simulink model "QC_Physics"  (R2026b)
settings: Solver=VariableStepAuto
undefined symbols (not defined in the file): N, Nm, rad, s, X, Y, Z
libraries: nesl_utility x13, sm_lib x5, simulink x1, fl_lib x1
settings Model: Creator=dani  LastModifiedBy=Dani

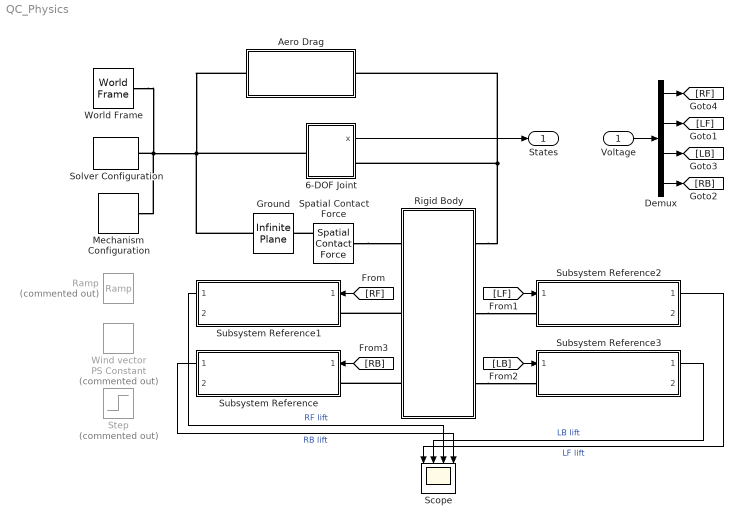
== system QC_Physics ==
  Voltage : Inport
  6-DOF Joint : Subsystem
  Aero Drag : Subsystem  ReferencedSubsystem=aero_drag
  Demux : Demux
  Ground : sm_lib/Curves and Surfaces/Infinite Plane  GraphicType=Rectangle  GraphicPlaneWidth=2  GraphicPlaneWidthUnits=m  GraphicPlaneHeight=2  GraphicPlaneHeightUnits=m  GraphicVisPropType=SimpleVisualProperties  GraphicDiffuseColor=[1 0.6667 0]  GraphicOpacity=0.4  GraphicSpecularColor=[0.5 0.5 0.5 1.0]  GraphicAmbientColor=[0.15 0.15 0.15 1.0]  GraphicEmissiveColor=[0.0 0.0 0.0 1.0]  GraphicShininess=75
  Mechanism Configuration : sm_lib/Utilities/Mechanism Configuration  UniformGravity=Constant  GravityVector=[0 0 -9.80665]  GravityVectorUnits=m/s^2  LinearizationDelta=0.001  JointModeTransitionNonlinearIterations=2
  Ramp : simulink/Sources/Ramp  Commented=on  slope=-715  start=0.37  InitialOutput=0
  Rigid Body : Subsystem  ReferencedSubsystem=rigid_body
  Scope : Scope  NumInputPorts=4
      settings: TimeSpan=1  ActiveDisplayString=4  ActiveDisplayYMinimum=-0.17596138261761787  ActiveDisplayYMaximum=1.5853977728105553  DataLoggingVariableName=ScopeData5
  Solver Configuration : nesl_utility/Solver Configuration  PhysicalDomain=network_engine_domain  SubClassName=solver  LeftPortType=input  RightPortType=generic  Tones=[]  Harmonics=[]  SimulateNoise=off  Profile=off  UseLocalSampling=off  EnableSwitchedLinearOptims=on  FrequencyDomain=off  UseCCode=off  RelTol=0.001  AbsTol=0.001  MinStep=1e-09  ToWorkspace=off  RevertToSquareIcSolve=off  NumHomotopyIterations=100  PhasorMode=off  PhasorModeNumHarmonics=1  ConsistencySolver=NEWTON_XTOL_AFTER_FTOL  CanonicalOrdering=UNORDERED  OptimizeIntermediates=UNOPTIMIZED  MulticoreSolverChoice=BACKWARD_EULER  IndexReductionMethod=DerivativeReplacement  DoDC=off  ResidualTolerance=1e-09  ConsistencyTolSource=GLOBAL  ConsistencyAbsTol=0.001  ConsistencyRelTol=0.001  ConsistencyTolFactor=0.001  UseLocalSolver=off  LocalSolverChoice=NE_BACKWARD_EULER_ADVANCER  ResolveIndetEquations=on  FunctionEvalNumThread=1  LocalSolverSampleTime=0.001  DoFixedCost=off  MaxNonlinIter=3  MaxModeIter=2  ComputeImpulses=off  ImpulseIterations=2  LinearAlgebra=auto  LinearAlgebraNumThread=0  EquationFormulation=NE_TIME_EF  DelaysMemoryBudget=1024  AutomaticFiltering=on  FilteringTimeConstant=0.001  PartitionStorageMethod=AS_NEEDED  PartitionMemoryBudget=1024  PartitionMethod=BALANCED  MultibodyUseLocalSolver=off  MultibodyLocalSolverChoice=ODE1  MultibodyLocalSolverSampleTime=0.001
  Spatial Contact Force : sm_lib/Forces and Torques/Spatial Contact Force  SenseSeparationDistance=on  NormalForceType=SmoothSpringDamper  NormalStiffness=1e3  NormalStiffnessUnits=N/m  NormalDamping=2e1  NormalDampingUnits=N/(m/s)  NormalTransitionRegionWidth=1e-3  NormalTransitionRegionWidthUnits=m  FrictionType=SmoothStickSlip  CoefficientOfStaticFriction=0.4  CoefficientOfDynamicFriction=0.4  FrictionalCriticalVelocity=1e-2  FrictionalCriticalVelocityUnits=m/s  SenseContactSignal=off  SensePenetrationDepth=off  SenseNormalVelocity=off  SenseTangentialVelocity=off  SensingForceTorqueDirection=BaseOnFollower  SensingForceTorqueResolutionFrame=ContactFrame  SenseNormalForce=off  SenseNormalForceMagnitude=off  SenseNormalTorque=off  SenseFrictionalForce=off  SenseFrictionalForceMagnitude=off  SenseFrictionalTorque=off  SenseTotalForce=off  SenseTotalTorque=off  SenseContactBaseRotation=off  SenseContactBaseTranslation=off  SenseContactFollowerRotation=off  SenseContactFollowerTranslation=off  ZeroCrossDetectContactStartAndEnd=on
  Step : Step  Commented=on  Time=2  FinalValue=4.1  SampleTime=0
  Subsystem Reference : Subsystem  ReferencedSubsystem=thruster  Dir=CCW  w2F=1e-3  w2F_u=N*s/rad  w2T=1e-5  w2T_u=Nm*s/rad  Color=[0 1 0]
  Subsystem Reference1 : Subsystem  ReferencedSubsystem=thruster  Dir=CW  w2F=1e-3  w2F_u=N*s/rad  w2T=1e-5  w2T_u=Nm*s/rad  Color=[1 0 0]
  Subsystem Reference2 : Subsystem  ReferencedSubsystem=thruster  Dir=CCW  w2F=1e-3  w2F_u=N*s/rad  w2T=1e-5  w2T_u=Nm*s/rad  Color=[0 1 0]
  Subsystem Reference3 : Subsystem  ReferencedSubsystem=thruster  Dir=CW  w2F=1e-3  w2F_u=N*s/rad  w2T=1e-5  w2T_u=Nm*s/rad  Color=[1 0 0]
  Wind vector : fl_lib/Physical Signals/Sources/PS Constant  Commented=on  constant=[1 0 0] m/s
  World Frame : sm_lib/Frames and Transforms/World Frame
  States : Outport
  wires:
  Demux/3 -> [LB]
  Demux/4 -> [RB]
  [RB] -> Subsystem Reference/1
  Subsystem Reference3/1 -> Scope/2  "LB lift"
  Subsystem Reference1/1 -> Scope/3  "RF lift"
  Voltage/1 -> Demux/1
  [LB] -> Subsystem Reference3/1
  Demux/1 -> [RF]
  [LF] -> Subsystem Reference2/1
  Subsystem Reference/1 -> Scope/4  "RB lift"
  [RF] -> Subsystem Reference1/1
  Subsystem Reference2/1 -> Scope/1  "LF lift"
  Demux/2 -> [LF]
  6-DOF Joint/1(x) -> States/1
  connections:
  6-DOF Joint/RConn1 -- Aero Drag/RConn1 -- Rigid Body/LConn1
  Solver Configuration/RConn1 -- Ground/LConn1 -- Aero Drag/LConn1 -- 6-DOF Joint/LConn1 -- World Frame/RConn1 -- Mechanism Configuration/RConn1
  Rigid Body/RConn3 -- Subsystem Reference/LConn1
  Rigid Body/LConn3 -- Subsystem Reference3/LConn1
  Spatial Contact Force/RConn1 -- Ground/RConn1
  Rigid Body/RConn2 -- Subsystem Reference1/LConn1
  Spatial Contact Force/LConn1 -- Rigid Body/RConn1
  Rigid Body/LConn2 -- Subsystem Reference2/LConn1

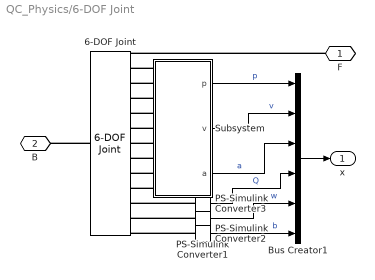
== system QC_Physics/6-DOF Joint ==
  6-DOF Joint : sm_lib/Joints/6-DOF Joint  JointMode=Normal  CompositeWrenchDir=FollowerOnBase  CompositeWrenchFrame=BaseFrame  SenseConstraintForce=off  SenseConstraintTorque=off  SenseTotalForce=off  SenseTotalTorque=off  PxPositionTargetSpecify=off  PxPositionTargetPriority=High  PxPositionTargetValue=0  PxPositionTargetValueUnits=m  PxVelocityTargetSpecify=off  PxVelocityTargetPriority=High  PxVelocityTargetValue=0  PxVelocityTargetValueUnits=m/s  PxEquilibriumPosition=0  PxEquilibriumPositionUnits=m  PxSpringStiffness=0  PxSpringStiffnessUnits=N/m  PxDampingCoefficient=0  PxDampingCoefficientUnits=N/(m/s)  PxLowerLimitSpecify=off  PxLowerLimitBound=-1  PxLowerLimitBoundUnits=m  PxLowerLimitStiffness=1e6  PxLowerLimitStiffnessUnits=N/m  PxLowerLimitDamping=1e3  PxLowerLimitDampingUnits=N/(m/s)  PxLowerLimitTransitionRegionWidth=1e-4  PxLowerLimitTransitionRegionWidthUnits=m  PxUpperLimitSpecify=off  PxUpperLimitBound=1  PxUpperLimitBoundUnits=m  PxUpperLimitStiffness=1e6  PxUpperLimitStiffnessUnits=N/m  PxUpperLimitDamping=1e3  PxUpperLimitDampingUnits=N/(m/s)  PxUpperLimitTransitionRegionWidth=1e-4  PxUpperLimitTransitionRegionWidthUnits=m  PxTorqueActuationMode=NoTorque  PxMotionActuationMode=ComputedMotion  PxSensePosition=on  PxSenseVelocity=on  PxSenseAcceleration=on  PxSenseTorqueForce=off  PxSenseLowerLimitTorqueForce=off  PxSenseUpperLimitTorqueForce=off  PyPositionTargetSpecify=off  PyPositionTargetPriority=High  PyPositionTargetValue=0  PyPositionTargetValueUnits=m  PyVelocityTargetSpecify=off  PyVelocityTargetPriority=High  PyVelocityTargetValue=0  PyVelocityTargetValueUnits=m/s  PyEquilibriumPosition=0  PyEquilibriumPositionUnits=m  PySpringStiffness=0  PySpringStiffnessUnits=N/m  PyDampingCoefficient=0  PyDampingCoefficientUnits=N/(m/s)  PyLowerLimitSpecify=off  PyLowerLimitBound=-1  PyLowerLimitBoundUnits=m  PyLowerLimitStiffness=1e6  PyLowerLimitStiffnessUnits=N/m  PyLowerLimitDamping=1e3  PyLowerLimitDampingUnits=N/(m/s)  PyLowerLimitTransitionRegionWidth=1e-4  PyLowerLimitTransitionRegionWidthUnits=m  PyUpperLimitSpecify=off  PyUpperLimitBound=1  PyUpperLimitBoundUnits=m  PyUpperLimitStiffness=1e6  PyUpperLimitStiffnessUnits=N/m  PyUpperLimitDamping=1e3  PyUpperLimitDampingUnits=N/(m/s)  PyUpperLimitTransitionRegionWidth=1e-4  PyUpperLimitTransitionRegionWidthUnits=m  PyTorqueActuationMode=NoTorque  PyMotionActuationMode=ComputedMotion  PySensePosition=on  PySenseVelocity=on  PySenseAcceleration=on  PySenseTorqueForce=off  PySenseLowerLimitTorqueForce=off  PySenseUpperLimitTorqueForce=off  PzPositionTargetSpecify=on  PzPositionTargetPriority=High  PzPositionTargetValue=350  PzPositionTargetValueUnits=mm  PzVelocityTargetSpecify=off  PzVelocityTargetPriority=High  PzVelocityTargetValue=0  PzVelocityTargetValueUnits=m/s  PzEquilibriumPosition=0  PzEquilibriumPositionUnits=m  PzSpringStiffness=0  PzSpringStiffnessUnits=N/m  PzDampingCoefficient=0  PzDampingCoefficientUnits=N/(m/s)  PzLowerLimitSpecify=off  PzLowerLimitBound=-1  PzLowerLimitBoundUnits=m  PzLowerLimitStiffness=1e6  PzLowerLimitStiffnessUnits=N/m  PzLowerLimitDamping=1e3  PzLowerLimitDampingUnits=N/(m/s)  PzLowerLimitTransitionRegionWidth=1e-4  PzLowerLimitTransitionRegionWidthUnits=m  PzUpperLimitSpecify=off  PzUpperLimitBound=1  PzUpperLimitBoundUnits=m  PzUpperLimitStiffness=1e6  PzUpperLimitStiffnessUnits=N/m  PzUpperLimitDamping=1e3  PzUpperLimitDampingUnits=N/(m/s)  PzUpperLimitTransitionRegionWidth=1e-4  PzUpperLimitTransitionRegionWidthUnits=m  PzTorqueActuationMode=NoTorque  PzMotionActuationMode=ComputedMotion  PzSensePosition=on  PzSenseVelocity=on  PzSenseAcceleration=on  PzSenseTorqueForce=off  PzSenseLowerLimitTorqueForce=off  PzSenseUpperLimitTorqueForce=off  SphPositionTargetSpecify=on  SphPositionTargetPriority=High  SphPositionTargetRotationMethod=RotationSequence  SphPositionTargetFollAlignAxisA=+X  SphPositionTargetBaseAlignAxisA=+Y  SphPositionTargetFollAlignAxisB=+Y  SphPositionTargetBaseAlignAxisB=+Z  SphPositionTargetRotationStandardAxis=+X  SphPositionTargetRotationAngle=30  SphPositionTargetRotationAngleUnits=deg  SphPositionTargetRotationArbitraryAxis=[0 0 1]  SphPositionTargetRotationSequenceAxes=FollowerAxes  SphPositionTargetRotationSequence=XYZ  SphPositionTargetRotationSequenceAngles=[10 2 0]*0  SphPositionTargetRotationSequenceAnglesUnits=deg  SphPositionTargetRotationMatrix=[1 0 0;0 1 0;0 0 1]  SphPositionTargetQuaternion=[1 0 0 0]  SphVelocityTargetSpecify=off  SphVelocityTargetPriority=High  SphVelocityTargetValue=[0 0 0]  SphVelocityTargetValueUnits=deg/s  SphVelocityTargetInFollowerFrame=on  SphEqPosRotationMethod=None  SphEqPosFollAlignAxisA=+X  SphEqPosBaseAlignAxisA=+Y  SphEqPosFollAlignAxisB=+Y  SphEqPosBaseAlignAxisB=+Z  SphEqPosRotationStandardAxis=+Z  SphEqPosRotationAngle=0  SphEqPosRotationAngleUnits=deg  SphEqPosRotationArbitraryAxis=[0 0 1]  SphEqPosRotationSequenceAxes=FollowerAxes  SphEqPosRotationSequence=XYX  SphEqPosRotationSequenceAngles=[0 0 0]  SphEqPosRotationSequenceAnglesUnits=deg  SphEqPosRotationMatrix=[1 0 0;0 1 0;0 0 1]  SphEqPosQuaternion=[1 0 0 0]  SphSpringStiffness=0  SphSpringStiffnessUnits=N*m/deg  SphDampingCoefficient=0  SphDampingCoefficientUnits=N*m/(deg/s)  SphLowerLimitSpecify=off  SphLowerLimitBound=15  SphLowerLimitBoundUnits=deg  SphLowerLimitStiffness=1e4  SphLowerLimitStiffnessUnits=N*m/deg  SphLowerLimitDamping=10  SphLowerLimitDampingUnits=N*m/(deg/s)  SphLowerLimitTransitionRegionWidth=0.1  SphLowerLimitTransitionRegionWidthUnits=deg  SphUpperLimitSpecify=off  SphUpperLimitBound=45  SphUpperLimitBoundUnits=deg  SphUpperLimitStiffness=1e4  SphUpperLimitStiffnessUnits=N*m/deg  SphUpperLimitDamping=10  SphUpperLimitDampingUnits=N*m/(deg/s)  SphUpperLimitTransitionRegionWidth=0.1  SphUpperLimitTransitionRegionWidthUnits=deg  SphTorqueActuationMode=NoTorque  SphActuateTorqueX=off  SphActuateTorqueY=off  SphActuateTorqueZ=off  SphActuateTorque=off  SphActuationFrame=BaseFrame  SphSensePosition=on  SphSenseVelocityX=off  SphSenseVelocityY=off  SphSenseVelocityZ=off  SphSenseVelocity=on  SphSenseAccelerationX=off  SphSenseAccelerationY=off  SphSenseAccelerationZ=off  SphSenseAcceleration=on  SphSenseLowerLimitTorqueMag=off  SphSenseUpperLimitTorqueMag=off  SphSensingFrame=BaseFrame
  Bus Creator1 : BusCreator  Inputs=6
  PS-Simulink Converter1 : nesl_utility/PS-Simulink Converter  PhysicalDomain=network_engine_domain  SubClassName=ps_output  LeftPortType=input  RightPortType=output  PseudoPeriodic=off  Frequencies=[]  VectorFormat=inherit  Unit=inherit  AffineConversion=off
  PS-Simulink Converter2 : nesl_utility/PS-Simulink Converter  PhysicalDomain=network_engine_domain  SubClassName=ps_output  LeftPortType=input  RightPortType=output  PseudoPeriodic=off  Frequencies=[]  VectorFormat=inherit  Unit=inherit  AffineConversion=off
  PS-Simulink Converter3 : nesl_utility/PS-Simulink Converter  PhysicalDomain=network_engine_domain  SubClassName=ps_output  LeftPortType=input  RightPortType=output  PseudoPeriodic=off  Frequencies=[]  VectorFormat=inherit  Unit=inherit  AffineConversion=off
  Subsystem : Subsystem
  F : PMIOPort  Side=Right
  B : PMIOPort  Port=2  Side=Left
  x : Outport
  wires:
  PS-Simulink Converter2/1 -> Bus Creator1/6  "b"
  PS-Simulink Converter1/1 -> Bus Creator1/5  "w"
  Subsystem/3(a) -> Bus Creator1/3  "a"
  Subsystem/2(v) -> Bus Creator1/2  "v"
  Subsystem/1(p) -> Bus Creator1/1  "p"
  Bus Creator1/1 -> x/1
  PS-Simulink Converter3/1 -> Bus Creator1/4  "Q"
  connections:
  PS-Simulink Converter2/LConn1 -- 6-DOF Joint/RConn13
  PS-Simulink Converter1/LConn1 -- 6-DOF Joint/RConn12
  Subsystem/LConn9 -- 6-DOF Joint/RConn10
  Subsystem/LConn8 -- 6-DOF Joint/RConn9
  Subsystem/LConn7 -- 6-DOF Joint/RConn8
  Subsystem/LConn6 -- 6-DOF Joint/RConn7
  Subsystem/LConn5 -- 6-DOF Joint/RConn6
  Subsystem/LConn4 -- 6-DOF Joint/RConn5
  Subsystem/LConn3 -- 6-DOF Joint/RConn4
  Subsystem/LConn2 -- 6-DOF Joint/RConn3
  Subsystem/LConn1 -- 6-DOF Joint/RConn2
  PS-Simulink Converter3/LConn1 -- 6-DOF Joint/RConn11
  F/RConn1 -- 6-DOF Joint/RConn1
  6-DOF Joint/LConn1 -- B/RConn1

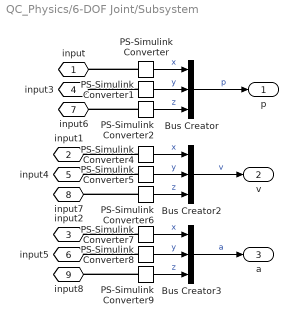
== system QC_Physics/6-DOF Joint/Subsystem ==
  Bus Creator : BusCreator  Inputs=3
  Bus Creator2 : BusCreator  Inputs=3
  Bus Creator3 : BusCreator  Inputs=3
  PS-Simulink Converter{,1..2,4..9} (9 alike) : nesl_utility/PS-Simulink Converter  PhysicalDomain=network_engine_domain  SubClassName=ps_output  LeftPortType=input  RightPortType=output  PseudoPeriodic=off  Frequencies=[]  VectorFormat=inherit  Unit=inherit  AffineConversion=off
  input : PMIOPort  Side=Left
  input1 : PMIOPort  Port=2  Side=Left
  input2 : PMIOPort  Port=3  Side=Left
  input3 : PMIOPort  Port=4  Side=Left
  input4 : PMIOPort  Port=5  Side=Left
  input5 : PMIOPort  Port=6  Side=Left
  input6 : PMIOPort  Port=7  Side=Left
  input7 : PMIOPort  Port=8  Side=Left
  input8 : PMIOPort  Port=9  Side=Left
  p : Outport
  v : Outport  Port=2
  a : Outport  Port=3
  wires:
  Bus Creator/1 -> p/1  "p"
  Bus Creator3/1 -> a/1  "a"
  PS-Simulink Converter8/1 -> Bus Creator3/2  "y"
  PS-Simulink Converter9/1 -> Bus Creator3/3  "z"
  PS-Simulink Converter7/1 -> Bus Creator3/1  "x"
  Bus Creator2/1 -> v/1  "v"
  PS-Simulink Converter5/1 -> Bus Creator2/2  "y"
  PS-Simulink Converter6/1 -> Bus Creator2/3  "z"
  PS-Simulink Converter4/1 -> Bus Creator2/1  "x"
  PS-Simulink Converter2/1 -> Bus Creator/3  "z"
  PS-Simulink Converter/1 -> Bus Creator/1  "x"
  PS-Simulink Converter1/1 -> Bus Creator/2  "y"
  connections:
  PS-Simulink Converter7/LConn1 -- input2/RConn1
  PS-Simulink Converter9/LConn1 -- input8/RConn1
  PS-Simulink Converter6/LConn1 -- input7/RConn1
  PS-Simulink Converter2/LConn1 -- input6/RConn1
  PS-Simulink Converter1/LConn1 -- input3/RConn1
  PS-Simulink Converter/LConn1 -- input/RConn1
  PS-Simulink Converter4/LConn1 -- input1/RConn1
  PS-Simulink Converter8/LConn1 -- input5/RConn1
  PS-Simulink Converter5/LConn1 -- input4/RConn1
